simulink model "New_VCU"  (R2023b)
settings: Solver=VariableStepAuto  StartTime=0.0  StopTime=10.0  RelTol=1e-3
undefined symbols (not defined in the file or in its folder): DiscIntNeverNeededParam
libraries: dspswit3 x2
settings Model: Creator=snith  LastModifiedBy=u32k60

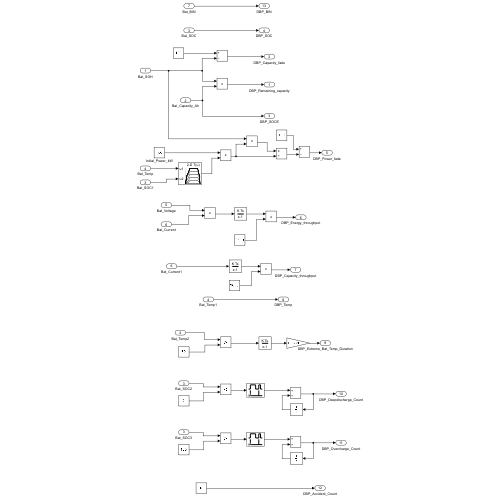
[thumbnail: Simulink's stored preview of the top-level diagram]
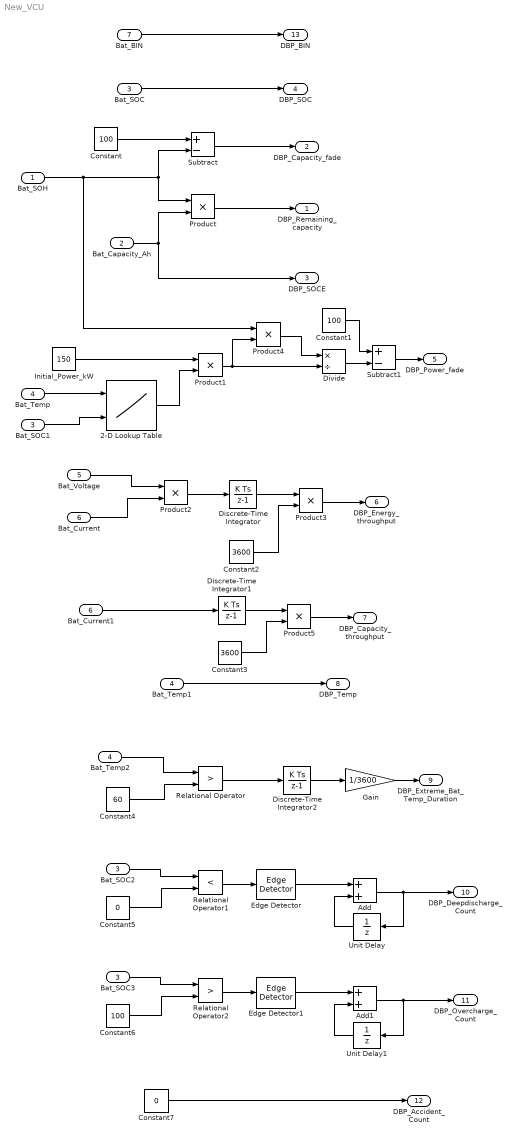
== system New_VCU ==
  Bat_SOH : Inport
  Bat_Capacity_Ah : Inport  Port=2
  Bat_SOC : Inport  Port=3
  Bat_Temp : Inport  Port=4
  Bat_Voltage : Inport  Port=5
  Bat_Current : Inport  Port=6
  Bat_BIN : Inport  Port=7
  2-D Lookup Table : Lookup_n-D  BreakpointsForDimension1=[-30;-20;-10;0;10;20;30;40;50;60;65]  BreakpointsForDimension2=[0;10;20;30;40;50;60;70;80;90;100]  Table=[0 0 0 0 0 0 0 0 0 0 0;0 0.05 0.1 0.2 0.4 0.5 0.5 0.5 0.5 0.5 0.5;0 0.1 0.2 0.4 0.6 0.75 0.75 0.75 0.75 0.75 0.75;0 0.2 0.4 0.6 0.8 1 1 1 1 1 1;0 0.2 0.4 0.6 0.8 1 1 1 1 1 1;0 0.2 0.4 0.6 0.8 1 1 1 1 1 1;0 0.2 0.4 0.6 0.8 1 1 1 1 1 1;0 0.2 0.4 0.6 0.8 1 1 1 1 1 1;0 0.2 0.4 0.6 0.8 1 1 1 1 1 1;0 0.1 0.2 0.4 0.6 0.5 0.5 0.5 0.5 0.5 0.5;0 0.05 0.1 0.2 0.4 0 0 0 0 0 0]  InternalRulePriority=Speed  RndMeth=Simplest
      settings: InputPortMap=u0,u1
  Add : Sum
  Add1 : Sum
  Bat_Current1 : InportShadow  Port=6
  Bat_SOC1 : InportShadow  Port=3
  Bat_SOC2 : InportShadow  Port=3
  Bat_SOC3 : InportShadow  Port=3
  Bat_Temp1 : InportShadow  Port=4
  Bat_Temp2 : InportShadow  Port=4
  Constant : Constant  Value=100
  Constant1 : Constant  Value=100
  Constant2 : Constant  Value=3600
  Constant3 : Constant  Value=3600
  Constant4 : Constant  Value=60
  Constant5 : Constant  Value=0
  Constant6 : Constant  Value=100
  Constant7 : Constant  Value=0
  Discrete-Time Integrator : DiscreteIntegrator  SampleTime=-1  ICPrevOutput=DiscIntNeverNeededParam  ICPrevScaledInput=DiscIntNeverNeededParam
  Discrete-Time Integrator1 : DiscreteIntegrator  SampleTime=-1  ICPrevOutput=DiscIntNeverNeededParam  ICPrevScaledInput=DiscIntNeverNeededParam
  Discrete-Time Integrator2 : DiscreteIntegrator  SampleTime=-1  ICPrevOutput=DiscIntNeverNeededParam  ICPrevScaledInput=DiscIntNeverNeededParam
  Divide : Product  Inputs=*/
  Edge Detector : dspswit3/Edge Detector  InputProcessing=Columns as channels (frame based)
  Edge Detector1 : dspswit3/Edge Detector  InputProcessing=Columns as channels (frame based)
  Gain : Gain  Gain=1/3600
  Initial_Power_kW : Constant  Value=150
  Product{,1..5} (6 alike) : Product
  Relational Operator : RelationalOperator  Operator=>  OutDataTypeStr=boolean  RndMeth=Simplest  InputSameDT=off
  Relational Operator1 : RelationalOperator  Operator=<  OutDataTypeStr=boolean  RndMeth=Simplest  InputSameDT=off
  Relational Operator2 : RelationalOperator  Operator=>  OutDataTypeStr=boolean  RndMeth=Simplest  InputSameDT=off
  Subtract : Sum  Inputs=+-
  Subtract1 : Sum  Inputs=+-
  Unit Delay : UnitDelay  SampleTime=-1  HasFrameUpgradeWarning=on
  Unit Delay1 : UnitDelay  SampleTime=-1  HasFrameUpgradeWarning=on
  DBP_Remaining_capacity : Outport
  DBP_Capacity_fade : Outport  Port=2
  DBP_SOCE : Outport  Port=3
  DBP_SOC : Outport  Port=4
  DBP_Power_fade : Outport  Port=5
  DBP_Energy_throughput : Outport  Port=6
  DBP_Capacity_throughput : Outport  Port=7
  DBP_Temp : Outport  Port=8
  DBP_Extreme_Bat_Temp_Duration : Outport  Port=9
  DBP_Deepdischarge_Count : Outport  Port=10
  DBP_Overcharge_Count : Outport  Port=11
  DBP_Accident_Count : Outport  Port=12
  DBP_BIN : Outport  Port=13
  wires:
  Bat_SOH/1 -> Product/1, Subtract/2, Product4/1
  Product/1 -> DBP_Remaining_capacity/1
  Constant/1 -> Subtract/1
  Subtract/1 -> DBP_Capacity_fade/1
  Bat_Capacity_Ah/1 -> Product/2, DBP_SOCE/1
  Bat_SOC/1 -> DBP_SOC/1
  Bat_Temp/1 -> 2-D Lookup Table/1
  Bat_SOC1/1 -> 2-D Lookup Table/2
  2-D Lookup Table/1 -> Product1/2
  Product1/1 -> Divide/2, Product4/2
  Bat_Voltage/1 -> Product2/1
  Bat_Current/1 -> Product2/2
  Product2/1 -> Discrete-Time Integrator/1
  Discrete-Time Integrator/1 -> Product3/1
  Constant2/1 -> Product3/2
  Product3/1 -> DBP_Energy_throughput/1
  Product5/1 -> DBP_Capacity_throughput/1
  Constant3/1 -> Product5/2
  Bat_Current1/1 -> Discrete-Time Integrator1/1
  Discrete-Time Integrator1/1 -> Product5/1
  Initial_Power_kW/1 -> Product1/1
  Product4/1 -> Divide/1
  Divide/1 -> Subtract1/2
  Constant1/1 -> Subtract1/1
  Subtract1/1 -> DBP_Power_fade/1
  Bat_Temp1/1 -> DBP_Temp/1
  Bat_Temp2/1 -> Relational Operator/1
  Constant4/1 -> Relational Operator/2
  Relational Operator/1 -> Discrete-Time Integrator2/1
  Discrete-Time Integrator2/1 -> Gain/1
  Gain/1 -> DBP_Extreme_Bat_Temp_Duration/1
  Bat_SOC2/1 -> Relational Operator1/1
  Constant5/1 -> Relational Operator1/2
  Relational Operator1/1 -> Edge Detector/1
  Edge Detector/1 -> Add/1
  Add/1 -> DBP_Deepdischarge_Count/1, Unit Delay/1
  Unit Delay/1 -> Add/2
  Constant6/1 -> Relational Operator2/2
  Add1/1 -> DBP_Overcharge_Count/1, Unit Delay1/1
  Unit Delay1/1 -> Add1/2
  Relational Operator2/1 -> Edge Detector1/1
  Edge Detector1/1 -> Add1/1
  Bat_SOC3/1 -> Relational Operator2/1
  Constant7/1 -> DBP_Accident_Count/1
  Bat_BIN/1 -> DBP_BIN/1
